simulink model "AngleTrackingInstancesTest"  (R2026b)
settings: Solver=FixedStepDiscrete  StopTime=0.03  FixedStep=pllA.Ts
PostLoadFcn:
  | addpath(fullfile(fileparts(get_param(bdroot,'FileName')),'..','build_process'));initialize_pll_instances(bdroot);
model workspace (MAT data in the model file):
  pllA.Ts = 5e-05
  pllA.NaturalFrequency = 40
  pllA.Damping = 0.707
  pllA.Kp = 100
  pllA.Ki = 0
  pllA.Kaw = 0
  pllA.OmegaMax = 1500
  pllA.MinMagnitude = 0.5
  pllA.LockError = 0.12
  pllA.LockSamples = 100
  pllA.Theta0 = -0.2
  pllA.Omega0 = 0
  pllB.Ts = 5e-05
  pllB.NaturalFrequency = 40
  pllB.Damping = 0.707
  pllB.Kp = 250
  pllB.Ki = 0
  pllB.Kaw = 0
  pllB.OmegaMax = 1500
  pllB.MinMagnitude = 0.5
  pllB.LockError = 0.12
  pllB.LockSamples = 100
  pllB.Theta0 = 0.3
  pllB.Omega0 = 0
libraries: AngleTracking x2
settings Model: Creator=24322  LastModifiedBy=24322

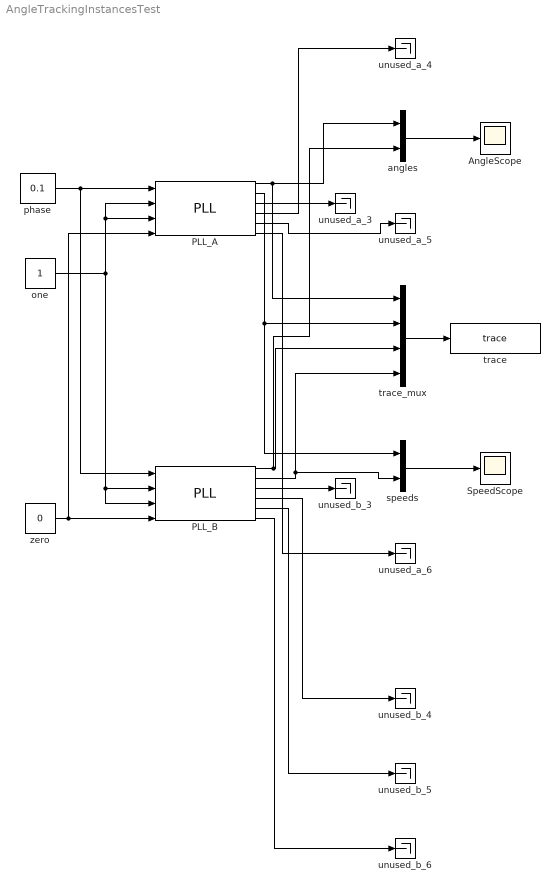
== system AngleTrackingInstancesTest ==
  AngleScope : Scope
  PLL_A : AngleTracking/PLL  pllCfg=pllA
  PLL_B : AngleTracking/PLL  pllCfg=pllB
  SpeedScope : Scope
  angles : Mux  Inputs=2
  one : Constant
  phase : Constant  Value=0.1
  speeds : Mux  Inputs=2
  trace : ToWorkspace  VariableName=trace  SaveFormat=Structure With Time  SampleTime=-1
  trace_mux : Mux
  unused_a_{3..6} (4 alike) : Terminator
  unused_b_{3..6} (4 alike) : Terminator
  zero : Constant  Value=0
  wires:
  speeds/1 -> SpeedScope/1
  angles/1 -> AngleScope/1
  trace_mux/1 -> trace/1
  PLL_B/6 -> unused_b_6/1
  PLL_B/5 -> unused_b_5/1
  PLL_B/4 -> unused_b_4/1
  PLL_B/3 -> unused_b_3/1
  PLL_B/2 -> trace_mux/4, speeds/2
  PLL_B/1 -> trace_mux/3, angles/2
  PLL_A/6 -> unused_a_6/1
  PLL_A/5 -> unused_a_5/1
  PLL_A/4 -> unused_a_4/1
  PLL_A/3 -> unused_a_3/1
  PLL_A/2 -> trace_mux/2, speeds/1
  PLL_A/1 -> trace_mux/1, angles/1
  zero/1 -> PLL_A/4, PLL_B/4
  one/1 -> PLL_B/2, PLL_B/3, PLL_A/2, PLL_A/3
  phase/1 -> PLL_A/1, PLL_B/1
